simulink model "dc_motor_supervisor"  (R2024b)
settings: Solver=FixedStepDiscrete  StartTime=0.0  StopTime=12  FixedStep=0.01  RelTol=1e-3  EnableMultiTasking=on
settings Model: Creator=Taha  LastModifiedBy=Taha
settings SolverCC: AlgebraicLoopSolver=TrustRegion  AutoInsertRateTranBlk=on
settings DataIOCC: LimitDataPoints=on
settings OptimizationCC: LifeSpan=inf
settings DebuggingCC: UnconnectedInputMsg=warning  UnconnectedOutputMsg=warning  UnconnectedLineMsg=warning  AllowSymbolicDim=off  SFUnexpectedBacktrackingDiag=warning  SFNoUnconditionalDefaultTransitionDiag=warning  SFExecutionAtInitializationDiag=none  ArithmeticOperatorsInVariantConditions=warning
settings ModelReferenceCC: EnableRefExpFcnMdlSchedulingChecks=on
settings SFSimCC: SimUseLocalCustomCode=off  CustomCodeUndefinedFunction=UseInterfaceOnly
settings RTWCC: RTWUseLocalCustomCode=off  GPUComputeCapability=3.5  DLArmComputeVersion=19.05
settings CodeAppCC: StateflowObjectComments=on
settings GRTTargetCC: TargetLangStandard=C89/C90 (ANSI)
settings ConfigComp: CovMetricSettings=dw  CovSaveCumulativeToWorkspaceVar=on  CovSaveSingleToWorkspaceVar=on  CovExternalEMLEnable=off  CovSFcnEnable=off

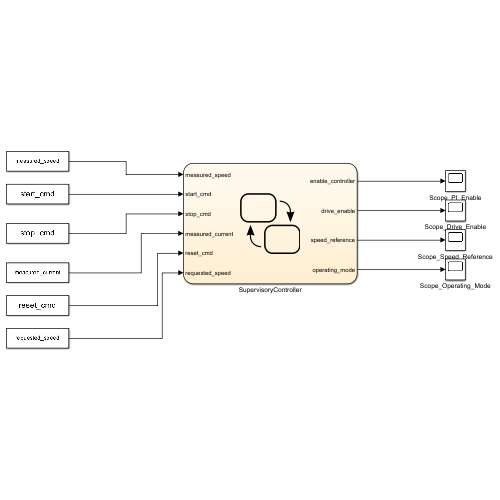
[thumbnail: Simulink's stored preview of the top-level diagram]
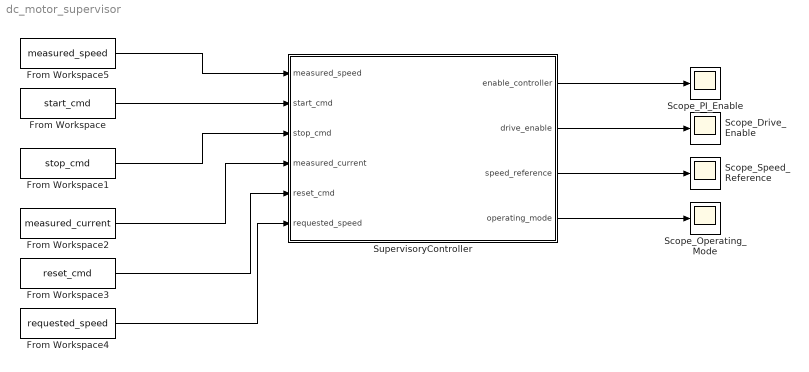
== system dc_motor_supervisor ==
  From Workspace : FromWorkspace  VariableName=start_cmd  Interpolate=off  OutputAfterFinalValue=Holding final value
  From Workspace1 : FromWorkspace  VariableName=stop_cmd  Interpolate=off  OutputAfterFinalValue=Holding final value
  From Workspace2 : FromWorkspace  VariableName=measured_current  Interpolate=off  OutputAfterFinalValue=Holding final value
  From Workspace3 : FromWorkspace  VariableName=reset_cmd  Interpolate=off  OutputAfterFinalValue=Holding final value
  From Workspace4 : FromWorkspace  VariableName=requested_speed  Interpolate=off  OutputAfterFinalValue=Setting to zero
  From Workspace5 : FromWorkspace  VariableName=measured_speed  Interpolate=off  OutputAfterFinalValue=Holding final value
  Scope_Drive_Enable : Scope
  Scope_Operating_Mode : Scope
  Scope_PI_Enable : Scope
  Scope_Speed_Reference : Scope
  SupervisoryController : Stateflow chart  TreatAsAtomicUnit=on
  wires:
  SupervisoryController/1(enable_controller) -> Scope_PI_Enable/1
  SupervisoryController/2(drive_enable) -> Scope_Drive_Enable/1
  SupervisoryController/3(speed_reference) -> Scope_Speed_Reference/1
  SupervisoryController/4(operating_mode) -> Scope_Operating_Mode/1
  From Workspace5/1 -> SupervisoryController/1(measured_speed)
  From Workspace/1 -> SupervisoryController/2(start_cmd)
  From Workspace1/1 -> SupervisoryController/3(stop_cmd)
  From Workspace2/1 -> SupervisoryController/4(measured_current)
  From Workspace3/1 -> SupervisoryController/5(reset_cmd)
  From Workspace4/1 -> SupervisoryController/6(requested_speed)

== stateflow chart dc_motor_supervisor/SupervisoryController ==
  settings: updateMethod=DISCRETE  sampleTime=0.01
  state IDLE
    entry:
    enable_controller = false;
    drive_enable = false;
    speed_reference = 0;
    operating_mode = uint8(0);
  state RUNNING
    entry:
    enable_controller = true;
    drive_enable = true;
    speed_reference = requested_speed;
    operating_mode = uint8(1);
    during:
    speed_reference = requested_speed;
  state STOPPING
    entry:
    enable_controller = true;
    drive_enable = true;
    speed_reference = 0;
    operating_mode = uint8(2);
  state FAULT
    entry:
    enable_controller = false;
    drive_enable = false;
    speed_reference = 0;
    operating_mode = uint8(3);
  (default) -> IDLE
  IDLE -> RUNNING [order 2] : [start_cmd && abs(measured_current) <= current_limit]
  RUNNING -> STOPPING [order 2] : [stop_cmd]
  FAULT -> IDLE : [reset_cmd && abs(measured_current) <= current_limit && ~start_cmd]
  IDLE -> FAULT [order 1] : [abs(measured_current) > current_limit]
  STOPPING -> IDLE [order 2] : [abs(measured_speed) < speed_tolerance]
  RUNNING -> FAULT [order 1] : [abs(measured_current) > current_limit]
  STOPPING -> FAULT [order 1] : [abs(measured_current) > current_limit]
  data: measured_speed input; start_cmd input; stop_cmd input; speed_tolerance local =0.02; measured_current input; current_limit local =0.5; reset_cmd input; enable_controller output boolean; drive_enable output boolean; speed_reference output double; operating_mode output uint8; requested_speed input double
